simulink model "Battery_Model_Order_first"  (R2025b)
settings: Solver=ode23t  StartTime=0.0  StopTime=500  MaxStep=0.01  RelTol=1e-3
libraries: fl_lib x8, nesl_utility x6, simulink x1
settings Model: Creator=psvan  LastModifiedBy=psvan

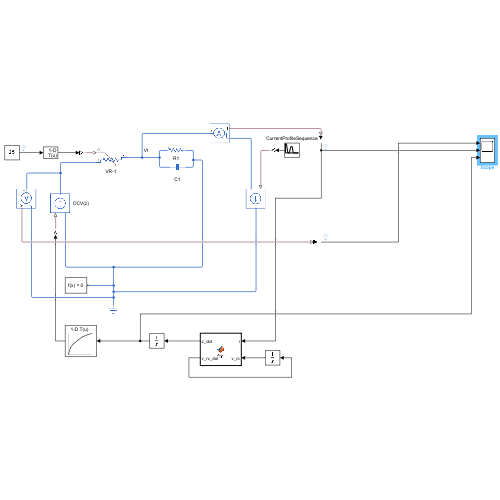
[thumbnail: Simulink's stored preview of the top-level diagram]
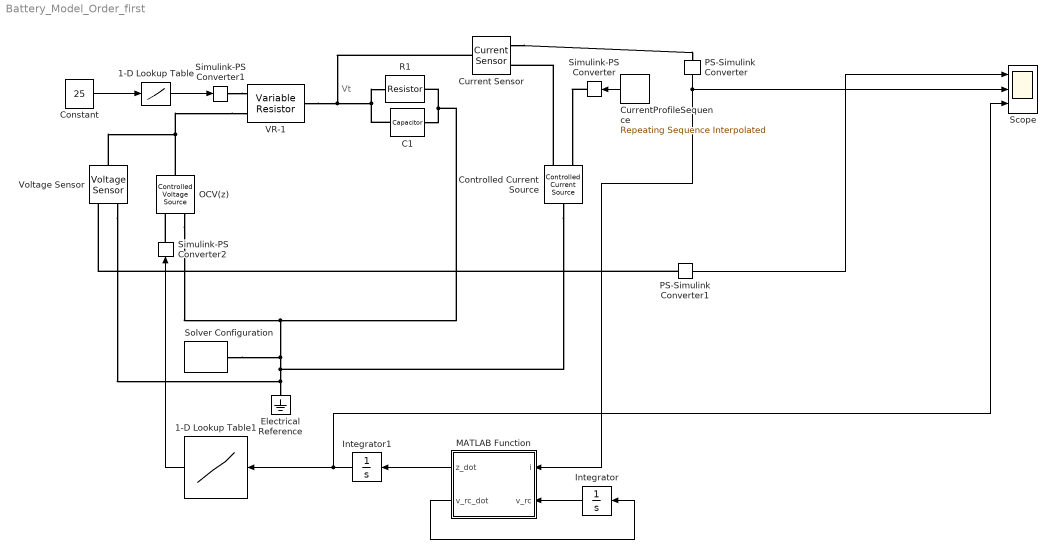
== system Battery_Model_Order_first ==
  note: Vt
  1-D Lookup Table : Lookup_n-D  NumberOfTableDimensions=1  BreakpointsForDimension1=[0, 25, 40]  Table=[0.019, 0.02, 0.021]  ExtrapMethod=Clip  InternalRulePriority=Speed  RndMeth=Simplest
  1-D Lookup Table1 : Lookup_n-D  NumberOfTableDimensions=1  BreakpointsForDimension1=[0 0.1 0.2 0.4 0.6 0.8 1]  Table=[3.0 3.4 3.6 3.8 4.0 4.1 4.2]  InternalRulePriority=Speed  RndMeth=Simplest
  C1 : fl_lib/Electrical/Electrical Elements/Capacitor  c=500 F  r=1e-6 Ohm  g=0 1/Ohm  i_specify=off  i_priority=None  i=0 A  i_nominal_specify=off  i_nominal_value=1  i_nominal_unit=A  v_specify=off  v_priority=None  v=0 V  v_nominal_specify=off  v_nominal_value=1  v_nominal_unit=V  vc_specify=off  vc_priority=High  vc=0 V  vc_nominal_specify=off  vc_nominal_value=1  vc_nominal_unit=V
  Constant : Constant  Value=25
  Controlled Current Source : fl_lib/Electrical/Electrical Sources/Controlled Current Source
  Current Sensor : fl_lib/Electrical/Electrical Sensors/Current Sensor
  CurrentProfileSequence : simulink/Sources/Repeating Sequence Interpolated  OutValues=[15 15 0 0 10 10 0 0]  TimeValues=[0 50 100 150 200 250 300 500]  LookUpMeth=Interpolation-Use End Values  tsamp=0.01  OutMin=[]  OutMax=[]  OutDataTypeStr=double  OutputDataTypeScalingMode=double  OutDataType=fixdt(0,8)  OutScaling=2^-10
  Electrical Reference : fl_lib/Electrical/Electrical Elements/Electrical Reference
  Integrator : Integrator
  Integrator1 : Integrator  InitialCondition=0.5
  MATLAB Function : MATLAB Function  TreatAsAtomicUnit=on
  OCV(z) : fl_lib/Electrical/Electrical Sources/Controlled Voltage Source
  PS-Simulink Converter : nesl_utility/PS-Simulink Converter  PhysicalDomain=network_engine_domain  SubClassName=ps_output  LeftPortType=input  RightPortType=output  PseudoPeriodic=off  Frequencies=[]  VectorFormat=inherit  Unit=inherit  AffineConversion=off
  PS-Simulink Converter1 : nesl_utility/PS-Simulink Converter  PhysicalDomain=network_engine_domain  SubClassName=ps_output  LeftPortType=input  RightPortType=output  PseudoPeriodic=off  Frequencies=[]  VectorFormat=inherit  Unit=inherit  AffineConversion=off
  R1 : fl_lib/Electrical/Electrical Elements/Resistor  R=0.01 Ohm  i_specify=off  i_priority=None  i=0 A  i_nominal_specify=off  i_nominal_value=1  i_nominal_unit=A  v_specify=off  v_priority=None  v=0 V  v_nominal_specify=off  v_nominal_value=1  v_nominal_unit=V
  Scope : Scope  NumInputPorts=3
      settings: ActiveDisplayYMinimum=-4.1392968767523648  ActiveDisplayYMaximum=15.226471411955179
  Simulink-PS Converter : nesl_utility/Simulink-PS Converter  PhysicalDomain=network_engine_domain  SubClassName=ps_input  LeftPortType=input  RightPortType=output  PseudoPeriodic=off  Frequencies=[]  NoiseDistribution=none  NoiseParameters=[]  Unit=1  AffineConversion=off  FilteringAndDerivatives=provide  SimscapeFilterOrder=1  InputFilterTimeConstant=0.001  UdotUserProvided=0
  Simulink-PS Converter1 : nesl_utility/Simulink-PS Converter  PhysicalDomain=network_engine_domain  SubClassName=ps_input  LeftPortType=input  RightPortType=output  PseudoPeriodic=off  Frequencies=[]  NoiseDistribution=none  NoiseParameters=[]  Unit=1  AffineConversion=off  FilteringAndDerivatives=provide  SimscapeFilterOrder=1  InputFilterTimeConstant=0.001  UdotUserProvided=0
  Simulink-PS Converter2 : nesl_utility/Simulink-PS Converter  PhysicalDomain=network_engine_domain  SubClassName=ps_input  LeftPortType=input  RightPortType=output  PseudoPeriodic=off  Frequencies=[]  NoiseDistribution=none  NoiseParameters=[]  Unit=1  AffineConversion=off  FilteringAndDerivatives=provide  SimscapeFilterOrder=1  InputFilterTimeConstant=0.001  UdotUserProvided=0
  Solver Configuration : nesl_utility/Solver Configuration  PhysicalDomain=network_engine_domain  SubClassName=solver  LeftPortType=input  RightPortType=generic  Tones=[]  Harmonics=[]  SimulateNoise=off  Profile=off  UseLocalSampling=off  EnableSwitchedLinearOptims=on  FrequencyDomain=off  UseCCode=off  RelTol=0.001  AbsTol=0.001  MinStep=1e-09  ToWorkspace=off  RevertToSquareIcSolve=off  NumHomotopyIterations=100  PhasorMode=off  PhasorModeNumHarmonics=1  ConsistencySolver=NEWTON_XTOL_AFTER_FTOL  IndexReductionMethod=DerivativeReplacement  DoDC=off  ResidualTolerance=1e-09  ConsistencyTolSource=GLOBAL  ConsistencyAbsTol=0.001  ConsistencyRelTol=0.001  ConsistencyTolFactor=0.001  UseLocalSolver=off  LocalSolverChoice=NE_BACKWARD_EULER_ADVANCER  ResolveIndetEquations=on  FunctionEvalNumThread=1  LocalSolverSampleTime=0.001  DoFixedCost=off  MaxNonlinIter=3  MaxModeIter=2  ComputeImpulses=off  ImpulseIterations=2  LinearAlgebra=auto  LinearAlgebraNumThread=0  EquationFormulation=NE_TIME_EF  DelaysMemoryBudget=1024  AutomaticFiltering=on  FilteringTimeConstant=0.001  PartitionStorageMethod=AS_NEEDED  PartitionMemoryBudget=1024  PartitionMethod=ROBUST  MultibodyUseLocalSolver=off  MultibodyLocalSolverChoice=ODE1  MultibodyLocalSolverSampleTime=0.001
  VR-1 : fl_lib/Electrical/Electrical Elements/Variable Resistor  Rmin=0.02 Ohm  thermalEnable=false  thermal_mass=1 J/K  i_specify=off  i_priority=None  i=0 A  i_nominal_specify=off  i_nominal_value=1  i_nominal_unit=A  v_specify=off  v_priority=None  v=0 V  v_nominal_specify=off  v_nominal_value=1  v_nominal_unit=V  T_specify=off  T_priority=None  T=300 K  T_nominal_specify=off  T_nominal_value=1  T_nominal_unit=K
  Voltage Sensor : fl_lib/Electrical/Electrical Sensors/Voltage Sensor
  wires:
  PS-Simulink Converter/1 -> Scope/2, MATLAB Function/1(i)
  Constant/1 -> 1-D Lookup Table/1
  MATLAB Function/2(v_rc_dot) -> Integrator/1
  1-D Lookup Table1/1 -> Simulink-PS Converter2/1
  MATLAB Function/1(z_dot) -> Integrator1/1
  Integrator1/1 -> Scope/3, 1-D Lookup Table1/1
  Integrator/1 -> MATLAB Function/2(v_rc)
  CurrentProfileSequence/1 -> Simulink-PS Converter/1
  PS-Simulink Converter1/1 -> Scope/1
  1-D Lookup Table/1 -> Simulink-PS Converter1/1
  connections:
  R1/LConn1 -- C1/LConn1 -- VR-1/RConn1 -- Current Sensor/LConn1
  VR-1/LConn2 -- OCV(z)/LConn1 -- Voltage Sensor/LConn1
  Electrical Reference/LConn1 -- Voltage Sensor/RConn2 -- Controlled Current Source/LConn1 -- C1/RConn1 -- R1/RConn1 -- OCV(z)/RConn2 -- Solver Configuration/RConn1
  PS-Simulink Converter1/LConn1 -- Voltage Sensor/RConn1
  Simulink-PS Converter1/RConn1 -- VR-1/LConn1
  Current Sensor/RConn1 -- PS-Simulink Converter/LConn1
  Simulink-PS Converter2/RConn1 -- OCV(z)/RConn1
  Simulink-PS Converter/RConn1 -- Controlled Current Source/RConn1
  Controlled Current Source/RConn2 -- Current Sensor/RConn2

== matlab function Battery_Model_Order_first/MATLAB Function ==
  data: i input; z_dot output; v_rc input; v_rc_dot output
function [z_dot, v_rc_dot] = fcn(i, v_rc)
Q = 3600;
eta = 0.995;
R1 = 0.01;
C1 = 500;
z_dot = -(eta * i) / Q; 
v_rc_dot = (i / C1) - (v_rc / (R1 * C1));
end
